simulink model "Input_delays"  (R2025a)
settings: Solver=VariableStepAuto  StartTime=0.0  StopTime=tf  RelTol=1e-3
values from neighbouring files (symbols this model uses):
  K = 1    [init.m]    (also in visu_m.m = evalin('base','K'))
  V0_vec = V0(:)    [init.m]
  W_mat = zeros(5)    [init.m]
  x_0 = [x1_0; v1_0;      x2_0; v2_0;      x3_0; v3_0;      x4_0; v4_0;      x5_0; v5_0]    [init.m]
settings Model: Creator=Lenovo  LastModifiedBy=Lenovo
settings DataIOCC: ReturnWorkspaceOutputs=off

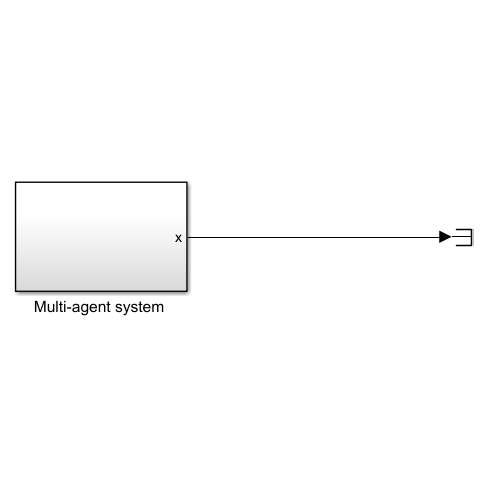
[thumbnail: Simulink's stored preview of the top-level diagram]
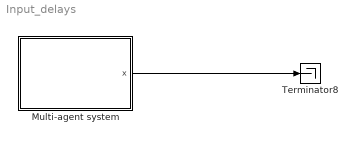
== system Input_delays ==
  "Multi-agent system " : Subsystem
  Terminator8 : Terminator
  wires:
  "Multi-agent system "/1(x) -> Terminator8/1

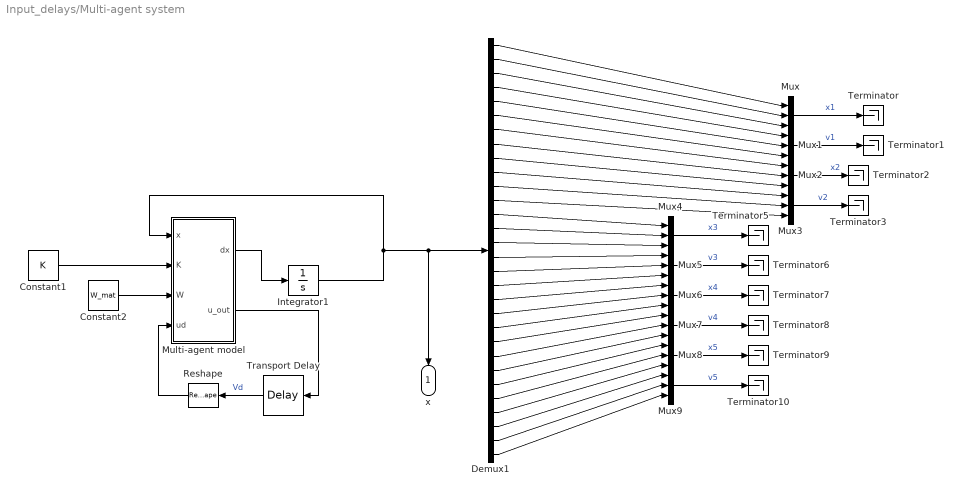
== system Input_delays/Multi-agent system  ==
  Constant1 : Constant  Value=K
  Constant2 : Constant  Value=W_mat  OutDataTypeStr=double
  Demux1 : Demux  Outputs=30
  Integrator1 : Integrator  InitialCondition=x_0
  Multi-agent model : MATLAB Function  TreatAsAtomicUnit=on
  Mux{,1..9} (10 alike) : Mux  Inputs=3
  Reshape : Reshape  OutputDimensionality=Customize  OutputDimensions=[3 5]
  Terminator{,1..3,5..10} (10 alike) : Terminator
  Transport Delay : TransportDelay  DelayTime=0.35  InitialOutput=V0_vec
  x : Outport  VectorParamsAs1DForOutWhenUnconnected=off
  wires:
  Mux/1 -> Terminator/1  "x1"
  Mux1/1 -> Terminator1/1  "v1"
  Demux1/1 -> Mux/1
  Demux1/2 -> Mux/2
  Demux1/3 -> Mux/3
  Demux1/4 -> Mux1/1
  Demux1/5 -> Mux1/2
  Demux1/6 -> Mux1/3
  Mux2/1 -> Terminator2/1  "x2"
  Demux1/7 -> Mux2/1
  Demux1/8 -> Mux2/2
  Demux1/9 -> Mux2/3
  Mux3/1 -> Terminator3/1  "v2"
  Demux1/10 -> Mux3/1
  Demux1/11 -> Mux3/2
  Demux1/12 -> Mux3/3
  Demux1/13 -> Mux4/1
  Demux1/14 -> Mux4/2
  Demux1/15 -> Mux4/3
  Demux1/16 -> Mux5/1
  Demux1/17 -> Mux5/2
  Demux1/18 -> Mux5/3
  Demux1/19 -> Mux6/1
  Demux1/20 -> Mux6/2
  Demux1/21 -> Mux6/3
  Demux1/22 -> Mux7/1
  Demux1/23 -> Mux7/2
  Demux1/24 -> Mux7/3
  Demux1/25 -> Mux8/1
  Demux1/26 -> Mux8/2
  Demux1/27 -> Mux8/3
  Demux1/28 -> Mux9/1
  Demux1/29 -> Mux9/2
  Demux1/30 -> Mux9/3
  Mux4/1 -> Terminator5/1  "x3"
  Mux5/1 -> Terminator6/1  "v3"
  Mux6/1 -> Terminator7/1  "x4"
  Mux7/1 -> Terminator8/1  "v4"
  Mux8/1 -> Terminator9/1  "x5"
  Mux9/1 -> Terminator10/1  "v5"
  Multi-agent model/1(dx) -> Integrator1/1
  Integrator1/1 -> x/1, Demux1/1, Multi-agent model/1(x)
  Constant2/1 -> Multi-agent model/3(W)
  Constant1/1 -> Multi-agent model/2(K)
  Transport Delay/1 -> Reshape/1  "Vd"
  Reshape/1 -> Multi-agent model/4(ud)
  Multi-agent model/2(u_out) -> Transport Delay/1

== matlab function Input_delays/Multi-agent system /Multi-agent model ==
  data: x input; K input; dx output; W input; ud input; u_out output
function [dx, u_out] = fcn(x,K,W,ud)

dx = zeros(30,1);

v1 = x(4:6);
v2 = x(10:12);
v3 = x(16:18);
v4 = x(22:24);
v5 = x(28:30);
V  = [v1,v2,v3,v4,v5];   

D = diag(sum(W,2));      

U = -K * ( V*D - V*W );  


u_out = U(:);           


dx(1:3)   = v1;
dx(7:9)   = v2;
dx(13:15) = v3;
dx(19:21) = v4;
dx(25:27) = v5;


dx(4:6)   = ud(:,1);
dx(10:12) = ud(:,2);
dx(16:18) = ud(:,3);
dx(22:24) = ud(:,4);
dx(28:30) = ud(:,5);
end
